simulink model "UBVM_Full_4Channel_System"  (R2023b)
settings: Solver=ode4  StopTime=150e-6  FixedStep=1e-8
Description:
  | Ultrasonic Bladder Volume Monitor - 4-Channel Multiplexed PZT + OPA357 + 5.88MHz LPF + MAX941 Comparator
settings Model: Creator=UBVM Engineering Suite

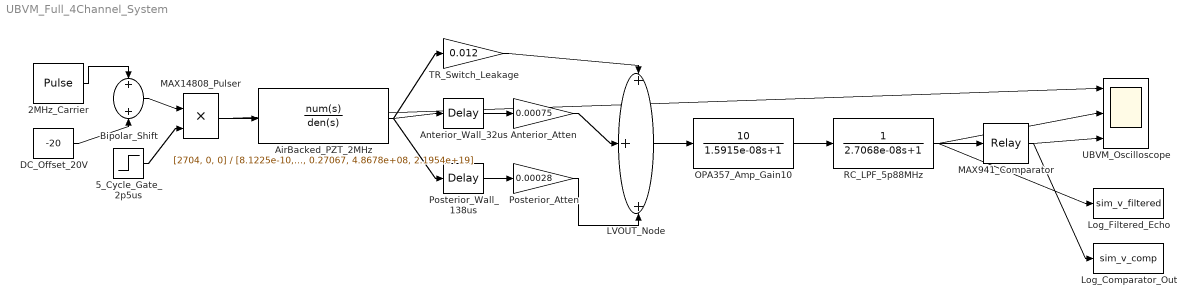
== system UBVM_Full_4Channel_System ==
  2MHz_Carrier : DiscretePulseGenerator  PulseType=Time based  Amplitude=40  Period=0.5e-6  PulseWidth=50
  DC_Offset_20V : Constant  Value=-20
  Bipolar_Shift : Sum  Inputs=++
  5_Cycle_Gate_2p5us : Step  Time=2.5e-6  Before=1  After=0
  MAX14808_Pulser : Product
  AirBacked_PZT_2MHz : TransferFcn  Numerator=[2704, 0, 0]  Denominator=[8.1225e-10, 2.964e-03, 0.27067, 4.8678e+08, 2.1954e+19]
  TR_Switch_Leakage : Gain  Gain=0.012
  Anterior_Wall_32us : TransportDelay  DelayTime=32e-6
  Anterior_Atten : Gain  Gain=0.00075
  Posterior_Wall_138us : TransportDelay  DelayTime=138e-6
  Posterior_Atten : Gain  Gain=0.00028
  LVOUT_Node : Sum  Inputs=+++
  OPA357_Amp_Gain10 : TransferFcn  Numerator=[10]  Denominator=[1.5915e-08, 1]
  RC_LPF_5p88MHz : TransferFcn  Numerator=[1]  Denominator=[2.7068e-08, 1]
  MAX941_Comparator : Relay  OnSwitchValue=0.038  OffSwitchValue=0.012  OnOutputValue=5.0  OffOutputValue=0.0
  UBVM_Oscilloscope : Scope  NumInputPorts=3
  Log_Filtered_Echo : ToWorkspace  VariableName=sim_v_filtered  SaveFormat=Array
  Log_Comparator_Out : ToWorkspace  VariableName=sim_v_comp  SaveFormat=Array
  wires:
  2MHz_Carrier/1 -> Bipolar_Shift/1
  DC_Offset_20V/1 -> Bipolar_Shift/2
  Bipolar_Shift/1 -> MAX14808_Pulser/1
  5_Cycle_Gate_2p5us/1 -> MAX14808_Pulser/2
  MAX14808_Pulser/1 -> AirBacked_PZT_2MHz/1
  MAX14808_Pulser/1 -> UBVM_Oscilloscope/1
  AirBacked_PZT_2MHz/1 -> TR_Switch_Leakage/1
  AirBacked_PZT_2MHz/1 -> Anterior_Wall_32us/1
  AirBacked_PZT_2MHz/1 -> Posterior_Wall_138us/1
  Anterior_Wall_32us/1 -> Anterior_Atten/1
  Posterior_Wall_138us/1 -> Posterior_Atten/1
  TR_Switch_Leakage/1 -> LVOUT_Node/1
  Anterior_Atten/1 -> LVOUT_Node/2
  Posterior_Atten/1 -> LVOUT_Node/3
  LVOUT_Node/1 -> OPA357_Amp_Gain10/1
  OPA357_Amp_Gain10/1 -> RC_LPF_5p88MHz/1
  RC_LPF_5p88MHz/1 -> MAX941_Comparator/1
  RC_LPF_5p88MHz/1 -> UBVM_Oscilloscope/2
  RC_LPF_5p88MHz/1 -> Log_Filtered_Echo/1
  MAX941_Comparator/1 -> UBVM_Oscilloscope/3
  MAX941_Comparator/1 -> Log_Comparator_Out/1
